simulink model "NanoBalancer_MotorTest"  (R2026b)
settings: Solver=daessc  StopTime=test_T  MaxStep=2e-5  RelTol=1e-4
PreLoadFcn:
  | InitNanoBalancer
InitFcn:
  | InitNanoBalancer
values from neighbouring files (symbols this model uses):
  test_T = 2.5    [run_NanoBalancer_MotorTest.m]
  test_u = 12    [run_NanoBalancer_MotorTest.m]
  test_wmax = 130    [run_NanoBalancer_MotorTest.m]
undefined symbols (not defined in the file or in its folder): GM
libraries: fl_lib x10, nesl_utility x7, simulink x3, ee_lib x2, sdl_lib x1, sl_discontinuities x1
settings Model: Creator=arkad  LastModifiedBy=arkad
settings SimscapeCC: SimscapeLogType=all  SimscapeNominalValues="[{\"value\":\"1\",\"unit\":\"A\"},{\"value\":\"1\",\"unit\":\"bar\"},{\"value\":\"1\",\"unit\":\"cm^2\"},{\"value\":\"1\",\"unit\":\"cm^3/s\"},{\"value\":\"1\",\"unit\":\"kJ/kg\"},{\"value\":\"1\",\"unit\":\"kW\"},{\"value\":\"1\",\"unit\":\"l\"},{\"value\":\"1\",\"unit\":\"N\"},{\"value\":\"1\",\"unit\":\"N*m\"},{\"value\":\"1\",\"unit\":\"V\"},{\"value\":\"0.001\",\"unit\":\"Wb\"}]"  SimscapeUseEnergyAccounting=off

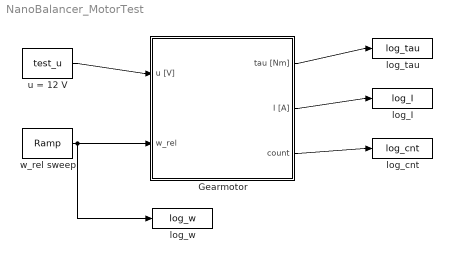
== system NanoBalancer_MotorTest ==
  Gearmotor : Subsystem
  log_I : ToWorkspace  VariableName=log_I  SaveFormat=Structure With Time  SampleTime=-1
  log_cnt : ToWorkspace  VariableName=log_cnt  SaveFormat=Structure With Time  SampleTime=-1
  log_tau : ToWorkspace  VariableName=log_tau  SaveFormat=Structure With Time  SampleTime=-1
  log_w : ToWorkspace  VariableName=log_w  SaveFormat=Structure With Time  SampleTime=-1
  u = 12 V : Constant  Value=test_u
  w_rel sweep : simulink/Sources/Ramp  slope=test_wmax/test_T  start=0  InitialOutput=0
  wires:
  u = 12 V/1 -> Gearmotor/1(u [V])
  w_rel sweep/1 -> Gearmotor/2(w_rel), log_w/1
  Gearmotor/1(tau [Nm]) -> log_tau/1
  Gearmotor/2(I [A]) -> log_I/1
  Gearmotor/3(count) -> log_cnt/1

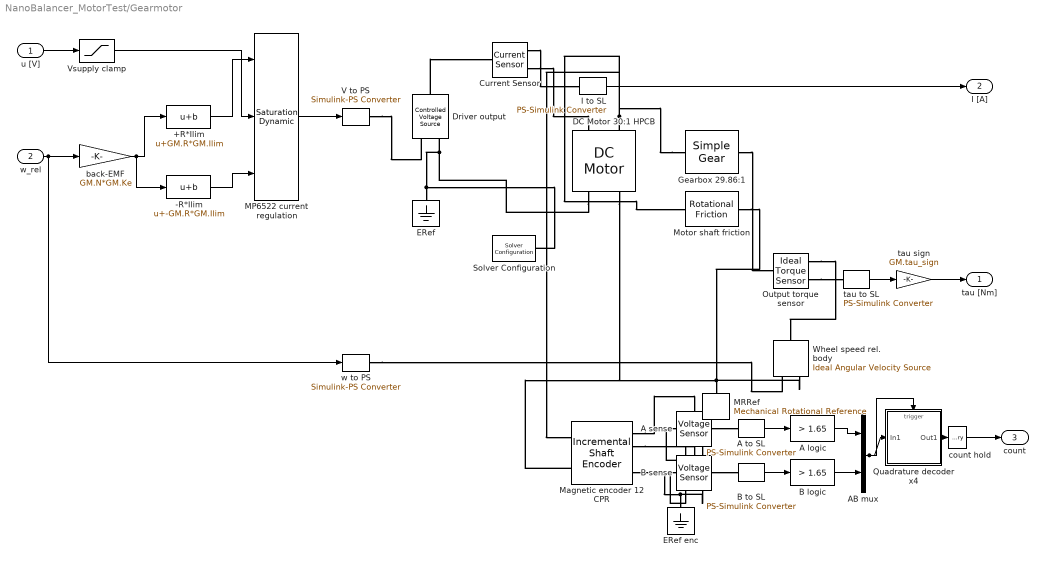
== system NanoBalancer_MotorTest/Gearmotor ==
  u [V] : Inport
  w_rel : Inport  Port=2
  +R*Ilim : Bias  Bias=GM.R*GM.Ilim  SaturateOnIntegerOverflow=off
  -R*Ilim : Bias  Bias=-GM.R*GM.Ilim  SaturateOnIntegerOverflow=off
  A logic : simulink/Logic and Bit Operations/Compare To Constant  relop=>  const=1.65  OutDataTypeStr=boolean
  A sense : fl_lib/Electrical/Electrical Sensors/Voltage Sensor
  A to SL : nesl_utility/PS-Simulink Converter  PhysicalDomain=network_engine_domain  SubClassName=ps_output  LeftPortType=input  RightPortType=output  PseudoPeriodic=off  Frequencies=[]  VectorFormat=inherit  Unit=inherit  AffineConversion=off
  AB mux : Mux  Inputs=2
  B logic : simulink/Logic and Bit Operations/Compare To Constant  relop=>  const=1.65  OutDataTypeStr=boolean
  B sense : fl_lib/Electrical/Electrical Sensors/Voltage Sensor
  B to SL : nesl_utility/PS-Simulink Converter  PhysicalDomain=network_engine_domain  SubClassName=ps_output  LeftPortType=input  RightPortType=output  PseudoPeriodic=off  Frequencies=[]  VectorFormat=inherit  Unit=inherit  AffineConversion=off
  Current Sensor : fl_lib/Electrical/Electrical Sensors/Current Sensor
  DC Motor 30:1 HPCB : ee_lib/Electromechanical/Brushed Motors/DC Motor  field_option=ee.enum.field_option.pm  Rf=100 Ohm  Lf=1 H  Laf=0.15 H  If0=0 A  parameterization=ee.enum.dcparam_option.circuit_param  Ra=GM.R Ohm  La=GM.La H  emf_or_torque=ee.enum.emf_or_torque.kv  Kv=GM.Ke V/(rad/s)  Ki=6.876e-4 N*m/A  T_stall=0.24e-3 N*m  w_max=19100 rpm  w_rated=15000 rpm  P_rated=0.08 W  V_rated=1.5 V  lam_param=ee.enum.lam_param.damping  i_noload=0 A  V_i_noload=1.5 V  J=GM.J_rotor kg*m^2  lam=0 N*m*s/rad  speed0=0 rpm  alpha=3.93e-3 1/K  Tmeas=25 degC  thermal_mass=100 J/K  initial_temperature=25 degC
  Driver output : fl_lib/Electrical/Electrical Sources/Controlled Voltage Source
  ERef : fl_lib/Electrical/Electrical Elements/Electrical Reference
  ERef enc : fl_lib/Electrical/Electrical Elements/Electrical Reference
  Gearbox 29.86:1 : sdl_lib/Gears/Simple Gear  ratio=GM.N  rotation_direction=1  friction_model=sdl.enum.gear_efficiencies_load.constant  T_noload=0.1 N*m  T_nom=5 N*m  efficiency_nom=0.8  efficiency=GM.eta_gb  temperature_TLU=[280, 300, 320] K  load_TLU=[1, 5, 10] N*m  efficiency_TLU=[.95, .9, .85]  efficiency_TLU2=[.85, .8, .75; .95, .9, .85; .85, .8, .7]  w_thr=0.5 rad/s  pwr_thr=0.001 W  enable_backlash=false  hardstop_model=simscape.enum.hardstop.smooth  backlash_distance=1e-3 mm  r_base=0.1 m  transition=1e-4 mm  backlash_stiffness=1e6 N/m  backlash_damping=1e3 N*s/m  coeff_rest=0.7  v_tol=0.001 m/s  f_tol=0.001 N  tau=0.1 s  mu_visc=[0, 0] N*m*s/rad  thermal_mass=50 J/K  temperature_specify=off  temperature_priority=High  temperature=300 K  temperature_nominal_specify=off  temperature_nominal_value=1  temperature_nominal_unit=K  x_backlash_specify=off  x_backlash_priority=None  x_backlash=0 mm  x_backlash_nominal_specify=off  x_backlash_nominal_value=1  x_backlash_nominal_unit=mm  f_hardstop_specify=off  f_hardstop_priority=None  f_hardstop=0 N  f_hardstop_nominal_specify=off  f_hardstop_nominal_value=1  f_hardstop_nominal_unit=N  v_backlash_specify=off  v_backlash_priority=None  v_backlash=0 m/s  v_backlash_nominal_specify=off  v_backlash_nominal_value=1  v_backlash_nominal_unit=m/s
  I to SL : nesl_utility/PS-Simulink Converter  PhysicalDomain=network_engine_domain  SubClassName=ps_output  LeftPortType=input  RightPortType=output  PseudoPeriodic=off  Frequencies=[]  VectorFormat=inherit  Unit=inherit  AffineConversion=off
  MP6522 current regulation : sl_discontinuities/Saturation Dynamic  OutMin=[]  OutMax=[]  OutDataTypeStr=Inherit: Same as second input  OutDataType=fixdt(1, 16)  OutScaling=2^-10  DoSatur=off
      settings: LibrarySourceBlock=|
      | simulink/Discontinuities/Saturation
      | Dynamic
  MRRef : fl_lib/Mechanical/Rotational Elements/Mechanical Rotational Reference
  Magnetic encoder 12 CPR : ee_lib/Sensors & Transducers/Incremental Shaft Encoder  NPulse=GM.PPR  Vm=3.3 V  angle0=1 deg
  Motor shaft friction : fl_lib/Mechanical/Rotational Elements/Rotational Friction  brkwy_trq=GM.Tc N*m  brkwy_vel=1 rad/s  Col_trq=GM.Tc N*m  visc_coef=0 N*m*s/rad  w_specify=off  w_priority=None  w=0 rad/s  w_nominal_specify=off  w_nominal_value=1  w_nominal_unit=rad/s  t_specify=off  t_priority=None  t=0 N*m  t_nominal_specify=off  t_nominal_value=1  t_nominal_unit=N*m
  Output torque sensor : fl_lib/Mechanical/Mechanical Sensors/Ideal Torque Sensor
  Quadrature decoder x4 : Subsystem  TreatAsAtomicUnit=on
  Solver Configuration : nesl_utility/Solver Configuration  PhysicalDomain=network_engine_domain  SubClassName=solver  LeftPortType=input  RightPortType=generic  Tones=[]  Harmonics=[]  SimulateNoise=off  Profile=off  UseLocalSampling=off  EnableSwitchedLinearOptims=on  FrequencyDomain=off  UseCCode=off  RelTol=0.001  AbsTol=0.001  MinStep=1e-09  ToWorkspace=off  RevertToSquareIcSolve=off  NumHomotopyIterations=100  PhasorMode=off  PhasorModeNumHarmonics=1  ConsistencySolver=NEWTON_XTOL_AFTER_FTOL  CanonicalOrdering=CANONICAL  OptimizeIntermediates=OPTIMIZED  MulticoreSolverChoice=BACKWARD_EULER  IndexReductionMethod=DerivativeReplacement  DoDC=off  ResidualTolerance=1e-09  ConsistencyTolSource=GLOBAL  ConsistencyAbsTol=0.001  ConsistencyRelTol=0.001  ConsistencyTolFactor=0.001  UseLocalSolver=off  LocalSolverChoice=NE_BACKWARD_EULER_ADVANCER  ResolveIndetEquations=on  FunctionEvalNumThread=1  LocalSolverSampleTime=0.001  DoFixedCost=off  MaxNonlinIter=3  MaxModeIter=2  ComputeImpulses=off  ImpulseIterations=2  LinearAlgebra=auto  LinearAlgebraNumThread=0  EquationFormulation=NE_TIME_EF  DelaysMemoryBudget=1024  AutomaticFiltering=on  FilteringTimeConstant=0.001  PartitionStorageMethod=AS_NEEDED  PartitionMemoryBudget=1024  PartitionMethod=BALANCED  MultibodyUseLocalSolver=off  MultibodyLocalSolverChoice=ODE1  MultibodyLocalSolverSampleTime=0.001
  V to PS : nesl_utility/Simulink-PS Converter  PhysicalDomain=network_engine_domain  SubClassName=ps_input  LeftPortType=input  RightPortType=output  PseudoPeriodic=off  Frequencies=[]  NoiseDistribution=none  NoiseParameters=[]  Unit=1  AffineConversion=off  FilteringAndDerivatives=provide  SimscapeFilterOrder=1  InputFilterTimeConstant=0.001  UdotUserProvided=0
  Vsupply clamp : Saturate  UpperLimit=GM.Vmax  LowerLimit=-GM.Vmax
  Wheel speed rel. body : fl_lib/Mechanical/Mechanical Sources/Ideal Angular Velocity Source
  back-EMF : Gain  Gain=GM.N*GM.Ke
  count hold : Memory
  tau sign : Gain  Gain=GM.tau_sign
  tau to SL : nesl_utility/PS-Simulink Converter  PhysicalDomain=network_engine_domain  SubClassName=ps_output  LeftPortType=input  RightPortType=output  PseudoPeriodic=off  Frequencies=[]  VectorFormat=inherit  Unit=inherit  AffineConversion=off
  w to PS : nesl_utility/Simulink-PS Converter  PhysicalDomain=network_engine_domain  SubClassName=ps_input  LeftPortType=input  RightPortType=output  PseudoPeriodic=off  Frequencies=[]  NoiseDistribution=none  NoiseParameters=[]  Unit=1  AffineConversion=off  FilteringAndDerivatives=filter  SimscapeFilterOrder=2  InputFilterTimeConstant=2e-4  UdotUserProvided=0
  tau [Nm] : Outport
  I [A] : Outport  Port=2
  count : Outport  Port=3
  wires:
  u [V]/1 -> Vsupply clamp/1
  w_rel/1 -> back-EMF/1, w to PS/1
  back-EMF/1 -> +R*Ilim/1, -R*Ilim/1
  +R*Ilim/1 -> MP6522 current regulation/1
  Vsupply clamp/1 -> MP6522 current regulation/2
  -R*Ilim/1 -> MP6522 current regulation/3
  MP6522 current regulation/1 -> V to PS/1
  tau to SL/1 -> tau sign/1
  tau sign/1 -> tau [Nm]/1
  I to SL/1 -> I [A]/1
  A to SL/1 -> A logic/1
  B to SL/1 -> B logic/1
  A logic/1 -> AB mux/1
  B logic/1 -> AB mux/2
  AB mux/1 -> Quadrature decoder x4/1(In1), Quadrature decoder x4/Trigger
  Quadrature decoder x4/1(Out1) -> count hold/1
  count hold/1 -> count/1
  connections:
  V to PS/RConn1 -- Driver output/RConn1
  Driver output/LConn1 -- Current Sensor/LConn1
  Current Sensor/RConn2 -- DC Motor 30:1 HPCB/LConn1
  Current Sensor/RConn1 -- I to SL/LConn1
  Driver output/RConn2 -- DC Motor 30:1 HPCB/RConn1 -- ERef/LConn1 -- Solver Configuration/RConn1
  Gearbox 29.86:1/LConn1 -- DC Motor 30:1 HPCB/LConn2 -- Motor shaft friction/LConn1 -- Magnetic encoder 12 CPR/LConn1
  Motor shaft friction/RConn1 -- DC Motor 30:1 HPCB/RConn2 -- Wheel speed rel. body/RConn2 -- MRRef/LConn1 -- Magnetic encoder 12 CPR/LConn2
  Gearbox 29.86:1/RConn1 -- Output torque sensor/LConn1
  Output torque sensor/RConn1 -- Wheel speed rel. body/LConn1
  w to PS/RConn1 -- Wheel speed rel. body/RConn1
  Output torque sensor/RConn2 -- tau to SL/LConn1
  Magnetic encoder 12 CPR/RConn4 -- A sense/RConn2 -- ERef enc/LConn1 -- B sense/RConn2
  Magnetic encoder 12 CPR/RConn1 -- A sense/LConn1
  Magnetic encoder 12 CPR/RConn2 -- B sense/LConn1
  A sense/RConn1 -- A to SL/LConn1
  B sense/RConn1 -- B to SL/LConn1

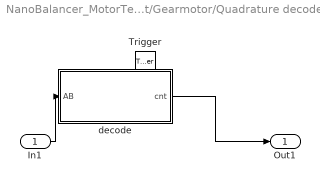
== system NanoBalancer_MotorTest/Gearmotor/Quadrature decoder x4 ==
  In1 : Inport
  Trigger : TriggerPort  TriggerType=either  VariantControl=(inherit)
  decode : MATLAB Function  TreatAsAtomicUnit=on
  Out1 : Outport  InitialOutput=0
  wires:
  In1/1 -> decode/1(AB)
  decode/1(cnt) -> Out1/1

== matlab function NanoBalancer_MotorTest/Gearmotor/Quadrature decoder x4/decode ==
  data: AB input size=[2 1]; cnt output
function cnt = decode(AB)
% x4 quadrature decoding: +1 per edge when A leads B (positive rotation)
persistent prev c
if isempty(prev), prev = 2*double(AB(1)) + double(AB(2)); c = 0; end
s = 2*double(AB(1)) + double(AB(2));
T = [0 -1 1 0; 1 0 0 -1; -1 0 0 1; 0 1 -1 0];
c = c + T(prev+1, s+1);
prev = s;
cnt = c;
